simulink model "HIL_MATLAB"  (R2024a)
settings: Solver=ode4  StartTime=0.0  StopTime=inf  FixedStep=0.005  RelTol=1e-3
undefined symbols (not defined in the file or in its folder): f
libraries: instrumentlib x2
settings Model: Creator=Houi  LastModifiedBy=ADMIN

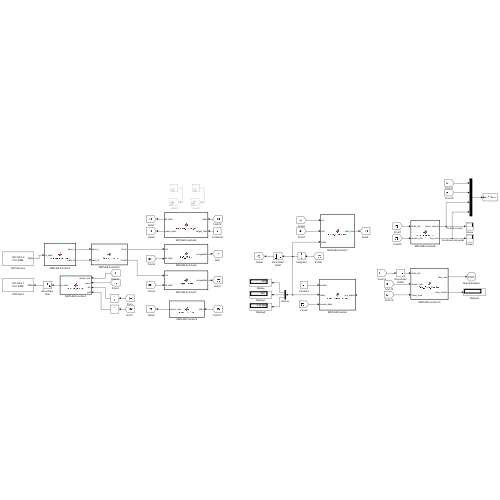
[thumbnail: Simulink's stored preview of the top-level diagram]
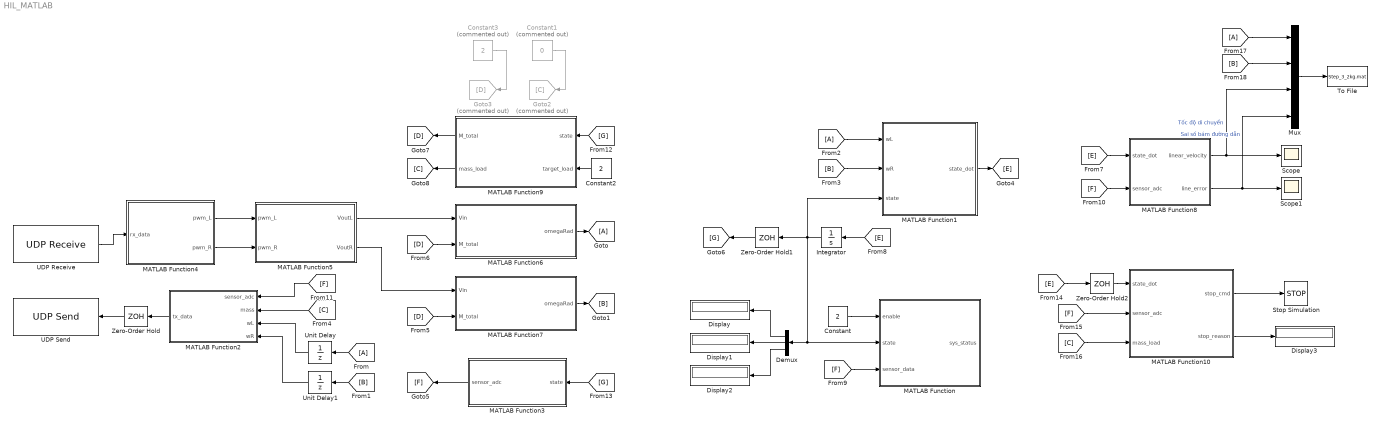
== system HIL_MATLAB ==
  Constant : Constant  Value=2
  Constant1 : Constant  Commented=on  Value=0
  Constant2 : Constant  Value=2
  Constant3 : Constant  Commented=on  Value=2
  Demux : Demux  Outputs=3
  Display{,1..3} (4 alike) : Display
  From : From
  From17 : From
  From2 : From
  Goto : Goto
  Goto2 : Goto  Commented=on  GotoTag=C
  Goto3 : Goto  Commented=on  GotoTag=D
  Integrator : Integrator  InitialCondition=[3000; 0; pi]
  MATLAB Function : MATLAB Function  TreatAsAtomicUnit=on
  MATLAB Function1 : MATLAB Function  TreatAsAtomicUnit=on
  MATLAB Function10 : MATLAB Function  TreatAsAtomicUnit=on
  MATLAB Function2 : MATLAB Function  TreatAsAtomicUnit=on
  MATLAB Function3 : MATLAB Function  TreatAsAtomicUnit=on
  MATLAB Function4 : MATLAB Function  TreatAsAtomicUnit=on
  MATLAB Function5 : MATLAB Function  TreatAsAtomicUnit=on
  MATLAB Function6 : MATLAB Function  TreatAsAtomicUnit=on
  MATLAB Function7 : MATLAB Function  TreatAsAtomicUnit=on
  MATLAB Function8 : MATLAB Function  TreatAsAtomicUnit=on
  MATLAB Function9 : MATLAB Function  TreatAsAtomicUnit=on
  Mux : Mux
  Scope : Scope
  Scope1 : Scope
  Stop Simulation : Stop
  To File : ToFile  Filename=Step_3_2kg.mat  SampleTime=0.005
  UDP Receive : instrumentlib/UDP Receive  Priority=2  LocalAddress=192.168.4.2  LocalPort=8888  EnablePortSharing=off  Host=192.168.4.1  Port=8889  GetLatestData=on  DataSize=[1 6]  DataType=uint8  ASCIIFormatting=%f,  Terminator=LF  CustomTerminator=10  ByteOrder=big-endian  EnableBlockingMode=on  Timeout=1  SampleTime=0.005  SimulateUsing=Interpreted execution
  UDP Send : instrumentlib/UDP Send  Priority=1  Host=192.168.4.1  Port=8889  LocalAddress=192.168.4.2  LocalPort=8888  EnablePortSharing=off  OutputDatagramPacketSize=512  ByteOrder=big-endian  EnableBlockingMode=off  SimulateUsing=Interpreted execution
  Unit Delay : UnitDelay  SampleTime=0.005  HasFrameUpgradeWarning=on
  Unit Delay1 : UnitDelay  SampleTime=0.005  HasFrameUpgradeWarning=on
  Zero-Order Hold : ZeroOrderHold  SampleTime=0.005
  Zero-Order Hold1 : ZeroOrderHold  SampleTime=0.005
  Zero-Order Hold2 : ZeroOrderHold  SampleTime=0.005
  wires:
  Constant/1 -> MATLAB Function/1(enable)
  MATLAB Function4/1(pwm_L) -> MATLAB Function5/1(pwm_L)
  MATLAB Function4/2(pwm_R) -> MATLAB Function5/2(pwm_R)
  MATLAB Function5/1(VoutL) -> MATLAB Function6/1(Vin)
  MATLAB Function5/2(VoutR) -> MATLAB Function7/1(Vin)
  MATLAB Function7/1(omegaRad) -> [B]
  MATLAB Function8/1(linear_velocity) -> Mux/3, Scope/1  "Tốc độ di chuyển"
  MATLAB Function8/2(line_error) -> Mux/4, Scope1/1  "Sai số bám đường dẫn"
  Demux/1 -> Display/1
  Demux/2 -> Display1/1
  Demux/3 -> Display2/1
  MATLAB Function2/1(tx_data) -> Zero-Order Hold/1
  UDP Receive/1 -> MATLAB Function4/1(rx_data)
  Zero-Order Hold/1 -> UDP Send/1
  Constant2/1 -> MATLAB Function9/2(target_load)
  From/1 -> Unit Delay/1
  [B] -> Unit Delay1/1
  MATLAB Function6/1(omegaRad) -> Goto/1
  From2/1 -> MATLAB Function1/1(wL)
  [B] -> MATLAB Function1/2(wR)
  [C] -> MATLAB Function2/2(mass)
  [D] -> MATLAB Function6/2(M_total)
  [D] -> MATLAB Function7/2(M_total)
  MATLAB Function1/1(state_dot) -> [E]
  [E] -> MATLAB Function8/1(state_dot)
  [E] -> Integrator/1
  MATLAB Function3/1(sensor_adc) -> [F]
  [F] -> MATLAB Function8/2(sensor_adc)
  [F] -> MATLAB Function2/1(sensor_adc)
  [G] -> MATLAB Function9/1(state)
  Integrator/1 -> MATLAB Function1/3(state), Demux/1, MATLAB Function/2(state), Zero-Order Hold1/1
  [G] -> MATLAB Function3/1(state)
  Zero-Order Hold1/1 -> [G]
  [F] -> MATLAB Function/3(sensor_data)
  [E] -> Zero-Order Hold2/1
  [F] -> MATLAB Function10/2(sensor_adc)
  [C] -> MATLAB Function10/3(mass_load)
  MATLAB Function10/2(stop_reason) -> Display3/1
  Zero-Order Hold2/1 -> MATLAB Function10/1(state_dot)
  Constant1/1 -> Goto2/1
  Constant3/1 -> Goto3/1
  MATLAB Function9/1(M_total) -> [D]
  MATLAB Function9/2(mass_load) -> [C]
  From17/1 -> Mux/1
  [B] -> Mux/2
  Mux/1 -> To File/1
  Unit Delay/1 -> MATLAB Function2/3(wL)
  Unit Delay1/1 -> MATLAB Function2/4(wR)
  MATLAB Function10/1(stop_cmd) -> Stop Simulation/1

== matlab function HIL_MATLAB/MATLAB Function1 ==
  data: wL input double size=1; wR input double size=1; state input double size=3; state_dot output double size=3
function state_dot = robot_kinematics(wL, wR, state)
    d = 190.0; % Khoang cach 2 banh chu dong B = 190 mm (Bảng 3.8)
    R = 32.5;  % Ban kinh banh xe D/2 = 32.5 mm (Bảng 3.4 & 3.8)
    theta = state(3);
    
    % Tinh van toc tinh tien (mm/s) va van toc goc (rad/s)
    v = (wR * R + wL * R) / 2.0;
    w = (wR * R - wL * R) / d;
    
    x_dot = v * cos(theta);
    y_dot = v * sin(theta);
    theta_dot = w;
    
    state_dot = [x_dot; y_dot; theta_dot];
end

== matlab function HIL_MATLAB/MATLAB Function ==
  settings: updateMethod=DISCRETE
  data: enable input; state input; sensor_data input; sys_status output
function sys_status = draw_environment(enable, state, sensor_data)
    coder.extrinsic('figure', 'hold', 'grid', 'axis', 'title', 'xlabel', ...
                    'ylabel', 'xlim', 'ylim', 'plot', 'text', 'rectangle', ...
                    'set', 'patch', 'drawnow', 'hgtransform', 'makehgtform', 'gca');
    
    persistent mapDrawn h_transform;
    sys_status = 1; 
    
    if enable == 0
        sys_status = 0; return;
    end
    
    %% 1. Khởi tạo sa bàn và Đối tượng Transform
    if isempty(mapDrawn) || isempty(h_transform)
        figure('Name', 'Simulation Environment', 'Color', 'w');
        hold on; grid on; axis equal;
        title('Sa ban xe do line'); 
        xlabel('X (mm)'); ylabel('Y (mm)');
        xlim([-200, 3200]); ylim([-500, 2000]);
        
        plot([3000, 500], [0, 0], 'k', 'LineWidth', 0.5);
        text(3000, -100, 'Bat dau', 'HorizontalAlignment', 'center');
        
        rectangle('Position', [850, -100, 300, 200], 'EdgeColor', 'r', 'LineStyle', '--', 'LineWidth', 0.5);
        text(1000, -200, 'Khu vuc tai hang', 'HorizontalAlignment', 'center');
        
        theta_R500 = linspace(-pi/2, pi/2, 100);
        plot(500 - 500 * cos(theta_R500), 500 - 500 * sin(theta_R500), 'k', 'LineWidth', 0.5);
        
        R = 800; alpha = acos(1 - (500 / (2 * R)));
        t1 = linspace(3*pi/2, 3*pi/2 + alpha, 50);
        x_S1 = 500 + R * cos(t1); y_S1 = 1800 + R * sin(t1);
        c2x = x_S1(end) + R * cos(pi/2 - alpha); c2y = y_S1(end) - R * sin(pi/2 - alpha);
        t2 = linspace(pi/2 + alpha, pi/2, 50);
        x_S2 = c2x + R * cos(t2); y_S2 = c2y + R * sin(t2);
        
        x_top = [x_S1, x_S2, 3000]; y_top = [y_S1, y_S2, y_S2(end)];
        plot(x_top, y_top, 'k', 'LineWidth', 0.5);
        text(3000, y_top(end) - 100, 'Ket thuc tren (1 kg)', 'HorizontalAlignment', 'center');
        
        y_bottom = 2000 - y_top;
        plot(x_top, y_bottom, 'k', 'LineWidth', 0.5);
        text(3000, y_bottom(end) + 100, 'Ket thuc duoi (2 kg)', 'HorizontalAlignment', 'center');
        
        % Tạo hệ trục tọa độ ảo cho robot
        h_transform = hgtransform('Parent', gca);
        
        % Chỉ vẽ vạch ngang trạm tải hàng (rộng 26 mm theo X, dài 50 mm theo Y)
        rectangle('Position', [1124, -25, 26, 50], 'FaceColor', 'k', 'EdgeColor', 'none');
        
        % Vẽ các bộ phận TẠI GỐC TỌA ĐỘ và gắn Parent vào h_transform
        patch('Parent', h_transform, 'XData', [-90, 90, 90, -90], 'YData', [-90, -90, 90, 90], 'FaceColor', 'b', 'EdgeColor', 'k'); 
        patch('Parent', h_transform, 'XData', [-20, 20, 20, -20], 'YData', [90, 90, 110, 110], 'FaceColor', 'r', 'EdgeColor', 'k'); 
        patch('Parent', h_transform, 'XData', [-20, 20, 20, -20], 'YData', [-110, -110, -90, -90], 'FaceColor', 'r', 'EdgeColor', 'k'); 
        % Sửa vị trí thanh cảm biến vẽ trên robot khớp X_sens = 75 mm
        patch('Parent', h_transform, 'XData', [70, 80, 80, 70], 'YData', [-35, -35, 35, 35], 'FaceColor', 'g', 'EdgeColor', 'k');
        
        mapDrawn = true;
    end
    
    %% 2. Cập nhật đồ họa
    if ~isempty(h_transform) && length(state) >= 3
        % Tính toán ma trận tịnh tiến và nội suy góc xoay Z
        T = makehgtform('translate', [state(1), state(2), 0], 'zrotate', state(3));
        
        % Áp dụng biến đổi cho toàn bộ khối thay vì từng mảng riêng lẻ
        set(h_transform, 'Matrix', T);
        
        % Bắt buộc xả bộ đệm đồ họa với giới hạn ~20 fps để ngăn nghẽn luồng Simulink
        drawnow limitrate; 
    end
    
    if max(sensor_data) < 150
        sys_status = 0; 
    end
end

== matlab function HIL_MATLAB/MATLAB Function2 ==
  data: sensor_adc input double size=[1 7]; tx_data output uint8 size=[1 21]; mass input double size=1; wL input double size=1; wR input double size=1
function tx_data = pack_udp_data(sensor_adc, mass, wL, wR)
    % 21-byte UDP packet from Simulink -> ESP32-S3 (200 Hz):
    % Byte 1     : Header 0xAA (170)
    % Bytes 2-15 : 7 x uint16 IR sensor ADC values (Little Endian, 0..1023)
    % Byte 16    : uint8 payload mass (0, 1, or 2 kg)
    % Bytes 17-18: int16 Left wheel linear velocity in mm/s (Little Endian)
    % Bytes 19-20: int16 Right wheel linear velocity in mm/s (Little Endian)
    % Byte 21    : uint8 XOR checksum of Bytes 2..20
    
    tx_data = zeros(1, 21, 'uint8');
    tx_data(1) = uint8(170); % 0xAA
    
    % Pack 7 ADC values (Bytes 2..15)
    for i = 1:7
        bytes = typecast(uint16(sensor_adc(i)), 'uint8');
        tx_data(2*i)     = bytes(1); % Low byte
        tx_data(2*i + 1) = bytes(2); % High byte
    end
    
    % Pack Mass (Byte 16)
    tx_data(16) = uint8(mass);
    
    % Convert angular velocity (rad/s) to linear velocity (mm/s) with R = 32.5 mm
    vL_mms = min(max(round(wL * 32.5), -32768), 32767);
    vR_mms = min(max(round(wR * 32.5), -32768), 32767);
    
    bytes_vL = typecast(int16(vL_mms), 'uint8');
    tx_data(17) = bytes_vL(1);
    tx_data(18) = bytes_vL(2);
    
    bytes_vR = typecast(int16(vR_mms), 'uint8');
    tx_data(19) = bytes_vR(1);
    tx_data(20) = bytes_vR(2);
    
    % Compute XOR Checksum (Byte 21)
    cs = uint8(0);
    for k = 2:20
        cs = bitxor(cs, tx_data(k));
    end
    tx_data(21) = cs;
end

== matlab function HIL_MATLAB/MATLAB Function3 ==
  settings: updateMethod=DISCRETE
  data: state input; sensor_adc output
function sensor_adc = read_sensors(state)
    persistent path_pts
    if isempty(path_pts)
        x1 = 3000:-1:500; y1 = zeros(1, length(x1));
        th = linspace(-pi/2, pi/2, 1500);
        x2 = 500 - 500*cos(th); y2 = 500 - 500*sin(th);

        x_S = linspace(500, 1661.8950, 1500);
        y_S1 = zeros(1, 1500); y_S2 = zeros(1, 1500);

        for i = 1:1500
            if x_S(i) < 1080.9475
                y_S1(i) = 1800 - sqrt(800^2 - (x_S(i) - 500)^2);
                y_S2(i) = 200  + sqrt(800^2 - (x_S(i) - 500)^2);
            else
                y_S1(i) = 700  + sqrt(800^2 - (x_S(i) - 1661.8950)^2);
                y_S2(i) = 1300 - sqrt(800^2 - (x_S(i) - 1661.8950)^2);
            end
        end
        x3_1 = [x_S, 1662:3000]; y3_1 = [y_S1, 1500*ones(1, length(1662:3000))];
        x3_2 = [x_S, 1662:3000]; y3_2 = [y_S2,  500*ones(1, length(1662:3000))];

        % Chỉ lưu đường tâm của line (không gộp meshgrid vạch ngang)
        path_pts = [x1, x2, x3_1, x3_2;
                    y1, y2, y3_1, y3_2];
    end

    x = state(1); y = state(2); theta = state(3);
    X_sens = 75.0;
    Y_sens = [30, 20, 10, 0, -10, -20, -30];

    % Thông số quang học: băng keo rộng 26 mm (nửa bề rộng 13 mm), h = 5 mm
    HALF_W      = 13.0;
    SIGMA_PSF   = 3.5;
    SQRT2_SIGMA = sqrt(2.0) * SIGMA_PSF;

    sensor_adc = zeros(1, 7);
    R_mat = [cos(theta), -sin(theta); sin(theta), cos(theta)];

    search_radius = 200.0;
    valid_idx = (path_pts(1,:) > x - search_radius) & (path_pts(1,:) < x + search_radius) & ...
                (path_pts(2,:) > y - search_radius) & (path_pts(2,:) < y + search_radius);
    local_path = path_pts(:, valid_idx);

    for i = 1:7
        coords = R_mat * [X_sens; Y_sens(i)];
        sens_x = x + coords(1);
        sens_y = y + coords(2);

        if isempty(local_path)
            min_dist = 1e6;
        else
            distances = (local_path(1,:) - sens_x).^2 + (local_path(2,:) - sens_y).^2;
            min_dist  = sqrt(min(distances));
        end

        % 1. Tích chập 1D erf cho băng keo rộng 26 mm + cắt mép vuông tại đích X = 3000 mm
        I_line = 0.5 * (erf((HALF_W - min_dist) / SQRT2_SIGMA) ...
                      + erf((HALF_W + min_dist) / SQRT2_SIGMA));
        I_end  = 0.5 * (1.0 + erf((3000.0 - sens_x) / SQRT2_SIGMA));
        I_line = I_line * I_end;

        % 2. Vạch ngang trạm tải hàng: X in [1124, 1150] mm, Y in [-25, 25] mm (không có vạch đích)
        I_bar_x = 0.5 * (erf((1150.0 - sens_x) / SQRT2_SIGMA) ...
                       - erf((1124.0 - sens_x) / SQRT2_SIGMA));
        I_bar_y = 0.5 * (erf((25.0   - sens_y) / SQRT2_SIGMA) ...
                       - erf((-25.0  - sens_y) / SQRT2_SIGMA));
        I_bar   = I_bar_x * I_bar_y;

        % Hợp vùng băng keo đen (bão hòa mức đen tối đa 1.0)
        I_opt = max(I_line, I_bar);

        % 3. Tiêm nhiễu trắng 20 ADC và lượng tử hóa 10-bit
        noisy_signal = 1023.0 * I_opt + 20.0 * randn();
        sensor_adc(i) = max(min(round(noisy_signal), 1023), 0);
    end
end

== matlab function HIL_MATLAB/MATLAB Function4 ==
  data: rx_data input uint8 size=[1 6]; pwm_L output double size=1; pwm_R output double size=1
function [pwm_L, pwm_R] = unpack_udp_data(rx_data)
    persistent last_pwm_L last_pwm_R;
    if isempty(last_pwm_L)
        last_pwm_L = 0.0;
        last_pwm_R = 0.0;
    end

    % Packet format (6 bytes uint8):
    % [0xBB, pwmL_low, pwmL_high, pwmR_low, pwmR_high, checksum]
    if numel(rx_data) >= 6 && rx_data(1) == uint8(187)
        cs = bitxor(bitxor(bitxor(rx_data(2), rx_data(3)), rx_data(4)), rx_data(5));
        if cs == rx_data(6)
            tempL = double(rx_data(2)) + double(rx_data(3)) * 256.0;
            if tempL > 32767.0
                tempL = tempL - 65536.0;
            end

            tempR = double(rx_data(4)) + double(rx_data(5)) * 256.0;
            if tempR > 32767.0
                tempR = tempR - 65536.0;
            end

            pwm_L = min(max(tempL / 100.0, -100.0), 100.0);
            pwm_R = min(max(tempR / 100.0, -100.0), 100.0);

            last_pwm_L = pwm_L;
            last_pwm_R = pwm_R;
        else
            pwm_L = last_pwm_L;
            pwm_R = last_pwm_R;
        end
    else
        pwm_L = last_pwm_L;
        pwm_R = last_pwm_R;
    end
end

== matlab function HIL_MATLAB/MATLAB Function5 ==
  data: pwm_L input double size=1; VoutL output double size=1; pwm_R input double size=1; VoutR output double size=1
function [VoutL, VoutR] = h_bridge_driver(pwm_L, pwm_R) 
    Vin = 12.0; 
    VoutL = Vin * (pwm_L / 100.0);
    VoutR = Vin * (pwm_R / 100.0);
end

== matlab function HIL_MATLAB/MATLAB Function6 ==
  data: Vin input double size=1; omegaRad output double size=1; M_total input double size=1
function omegaRad = Left_Motor(Vin, M_total)
    persistent omega_prev;
    if isempty(omega_prev)
        omega_prev = 0.0;
    end
    
    u_in = double(Vin(1));
    m_tot = double(M_total(1));
    
    % --- 1. Identified Bench Parameters (JGB37-520 333 RPM + 65mm Wheel) ---
    Ts = 0.005;             % Sampling period = 0.005s (200 Hz)
    K_dc_omega = 2.9736;    % Steady-state gain (rad/s per Volt)
    tau_0 = 0.055;          % Bench mechanical time constant with wheel in air (s)
    V_deadzone_0 = 0.252;   % Unloaded static friction deadzone (2.10% PWM * 12V)
    
    % --- 2. Variable-Mass Coupling ---
    gamma_inertia = 0.0384; % Time-constant increase per kg of total mass (s/kg)
    k_V_roll = 0.186;       % Rolling + slope friction voltage drop per kg (V/kg)
    
    tau_eff = tau_0 + gamma_inertia * m_tot;
    V_thresh = V_deadzone_0 + k_V_roll * m_tot;
    
    % --- 3. Friction & TB6612FNG Short-Brake Physics ---
    if abs(omega_prev) < 0.05
        if abs(u_in) <= V_thresh
            V_eff = 0.0;
            omega_prev = 0.0;
        else
            V_eff = u_in - sign(u_in) * V_thresh;
        end
    else
        V_eff = u_in - sign(omega_prev) * V_thresh;
    end
    
    % --- 4. Exact ZOH Discrete-Time Transfer Function Update ---
    alpha_d = exp(-Ts / tau_eff);
    omega_new = alpha_d * omega_prev + (1.0 - alpha_d) * (K_dc_omega * V_eff);
    
    if abs(u_in) <= V_thresh && (omega_new * omega_prev <= 0.0 || abs(omega_new) < 0.05)
        omega_new = 0.0;
    end
    
    omega_prev = omega_new;
    omegaRad = omega_new;
end

== matlab function HIL_MATLAB/MATLAB Function7 ==
  data: Vin input double size=1; omegaRad output double size=1; M_total input double size=1
function omegaRad = Right_Motor(Vin, M_total)
    persistent omega_prev;
    if isempty(omega_prev)
        omega_prev = 0.0;
    end
    
    u_in = double(Vin(1));
    m_tot = double(M_total(1));
    
    % --- 1. Identified Bench Parameters (JGB37-520 333 RPM + 65mm Wheel) ---
    Ts = 0.005;             % Sampling period = 0.005s (200 Hz)
    K_dc_omega = 2.9736;    % Steady-state gain (rad/s per Volt)
    tau_0 = 0.055;          % Bench mechanical time constant with wheel in air (s)
    V_deadzone_0 = 0.252;   % Unloaded static friction deadzone (2.10% PWM * 12V)
    
    % --- 2. Variable-Mass Coupling ---
    gamma_inertia = 0.0384; % Time-constant increase per kg of total mass (s/kg)
    k_V_roll = 0.186;       % Rolling + slope friction voltage drop per kg (V/kg)
    
    tau_eff = tau_0 + gamma_inertia * m_tot;
    V_thresh = V_deadzone_0 + k_V_roll * m_tot;
    
    % --- 3. Friction & TB6612FNG Short-Brake Physics ---
    if abs(omega_prev) < 0.05
        if abs(u_in) <= V_thresh
            V_eff = 0.0;
            omega_prev = 0.0;
        else
            V_eff = u_in - sign(u_in) * V_thresh;
        end
    else
        V_eff = u_in - sign(omega_prev) * V_thresh;
    end
    
    % --- 4. Exact ZOH Discrete-Time Transfer Function Update ---
    alpha_d = exp(-Ts / tau_eff);
    omega_new = alpha_d * omega_prev + (1.0 - alpha_d) * (K_dc_omega * V_eff);
    
    if abs(u_in) <= V_thresh && (omega_new * omega_prev <= 0.0 || abs(omega_new) < 0.05)
        omega_new = 0.0;
    end
    
    omega_prev = omega_new;
    omegaRad = omega_new;
end

== matlab function HIL_MATLAB/MATLAB Function8 ==
  data: state_dot input; linear_velocity output; sensor_adc input; line_error output
function [linear_velocity, line_error] = Data_Processor(state_dot, sensor_adc)
    % 1. Tính tốc độ dài (mm/s)
    % state_dot = [vx, vy, omega]
    linear_velocity = sqrt(state_dot(1)^2 + state_dot(2)^2);
    
    % 2. Tính sai số e_y (mm) - Tái hiện logic của STM32
    weights = [30, 20, 10, 0, -10, -20, -30];
    sum_adc = sum(sensor_adc);
    
    if sum_adc > 0
        line_error = sum(sensor_adc .* weights) / sum_adc;
    else
        line_error = 0; % Hoặc giữ giá trị cuối cùng
    end
end

== matlab function HIL_MATLAB/MATLAB Function9 ==
  data: state input double size=3; M_total output double size=1; target_load input double size=1; mass_load output double size=1
function [M_total, mass_load] = Payload_Manager(state, target_load)
    % Empty robot mass m_xe = 2.0 kg (Table 3.7 MechanicalDesign.docx)
    m_xe = 2.0;
    
    persistent has_loaded;
    if isempty(has_loaded)
        has_loaded = false;
    end
    
    x = state(1);
    y = state(2);
    
    % Loading zone rectangle: X in [850, 1150] mm, Y in [-100, 100] mm
    if (x >= 850.0 && x <= 1150.0 && abs(y) <= 100.0)
        has_loaded = true;
    end
    
    if has_loaded
        mass_load = double(target_load);
    else
        mass_load = 0.0;
    end
    
    M_total = m_xe + mass_load;
end

== matlab function HIL_MATLAB/MATLAB Function10 ==
  data: state_dot input double size=[3 1]; stop_cmd output; sensor_adc input double size=[1 7]; mass_load input double size=1; stop_reason output
function [stop_cmd, stop_reason] = Sim_Stop_Monitor(state_dot, sensor_adc, mass_load)
% stop_reason:
%   0 = Đang chạy
%   1 = Dừng thành công tại đích (đứng yên liên tục >= 2.0 s sau khi chở tải > 4.0 m)
%   2 = Mất tín hiệu bám line e2 liên tục >= 2.0 s

    persistent goal_dwell_t line_loss_t dist_after_load_mm
    if isempty(goal_dwell_t)
        goal_dwell_t       = 0.0;
        line_loss_t        = 0.0;
        dist_after_load_mm = 0.0;
    end

    Ts = 0.005; % Khớp Zero-Order Hold2 (200 Hz)

    % Vận tốc tịnh tiến [mm/s] từ state_dot = [x_dot; y_dot; theta_dot]
    v_mms = hypot(double(state_dot(1)), double(state_dot(2)));

    % Tích lũy quãng đường sau khi đã nhận tải tại trạm (phân biệt trạm tải vs đích)
    if mass_load > 0
        dist_after_load_mm = dist_after_load_mm + v_mms * Ts;
    end

    % Kiểm tra còn tín hiệu e2 hợp lệ (đồng bộ ngưỡng total_I >= 0.15 của app.c)
    norm_adc = double(sensor_adc) / 1023.0 - 0.085;
    norm_adc(norm_adc < 0.02) = 0.0;
    line_present = (sum(norm_adc) >= 0.15);

    % 1) Đang đứng yên tại đích: đã mang tải, đi > 4000 mm sau trạm tải và v < 5 mm/s
    at_goal_standstill = (mass_load > 0) && (dist_after_load_mm > 4000.0) && (v_mms < 5.0);

    if at_goal_standstill
        goal_dwell_t = goal_dwell_t + Ts;
        line_loss_t  = 0.0; % Không tính là mất line khi đã dừng gọn ở đích (X_sens = 3075)
    else
        goal_dwell_t = 0.0;
        if ~line_present
            line_loss_t = line_loss_t + Ts;
        else
            line_loss_t = 0.0;
        end
    end

    stop_cmd    = 0;
    stop_reason = 0;

    if goal_dwell_t >= 2.0
        stop_cmd    = 1;
        stop_reason = 1;
    elseif line_loss_t >= 2.0
        stop_cmd    = 1;
        stop_reason = 2;
    end
end
